simulink model "StratifiedHotWaterStorageTank"  (R2025a)
settings: Solver=VariableStepAuto  StartTime=0.0  StopTime=3600  RelTol=1e-3  AbsTol=1e-3
PreLoadFcn:
  | tankHeight = 1.6;
  | tankVolume = 0.2;
  | numberLayers = 8;
  | upwardConvectionCoeff = 50000;
  | downwardConvectionCoeff = 5;
libraries: fl_lib x30, nesl_utility x5, SimscapeFluids_lib x1
CloseFcn:
  | try, close(h1_StratifiedHotWaterStorageTank), end
  | clear h1_StratifiedHotWaterStorageTank
  | try, close(h2_StratifiedHotWaterStorageTank), end
  | clear h2_StratifiedHotWaterStorageTank
  | 
  | clear simlog_StratifiedHotWaterStorageTank
  | clear tankVolume tankHeight numberLayers upwardConvectionCoeff downwardConvectionCoeff
Description:
  | Stratified Hot Water Storage Tank
settings Model: Creator=The MathWorks, Inc.  LastModifiedBy=The MathWorks, Inc.
settings SolverCC: AutoScaleAbsTol=off  MaxConsecutiveMinStep=3  AlgebraicLoopSolver=TrustRegion  MaxZcPerStep=1.0
settings DataIOCC: SaveOutput=off  SignalLogging=off  DSMLogging=off  SaveTime=off  ReturnWorkspaceOutputs=off
settings DebuggingCC: UnconnectedInputMsg=warning  UnconnectedOutputMsg=warning  UnconnectedLineMsg=warning  SymbolicDimsDataTypeCodeGenerationDiagnostic=none
settings ModelReferenceCC: EnableRefExpFcnMdlSchedulingChecks=on
settings SFSimCC: CustomCodeUndefinedFunction=UseInterfaceOnly
settings RTWCC: GPUComputeCapability=3.5  DLArmComputeVersion=19.05
settings SimscapeCC: SimscapeLogType=all  SimscapeLogSimulationStatistics=on  SimscapeLogName=simlog_StratifiedHotWaterStorageTank  SimscapeLogLimitData=off  SimscapeLogDataHistory=10000.0

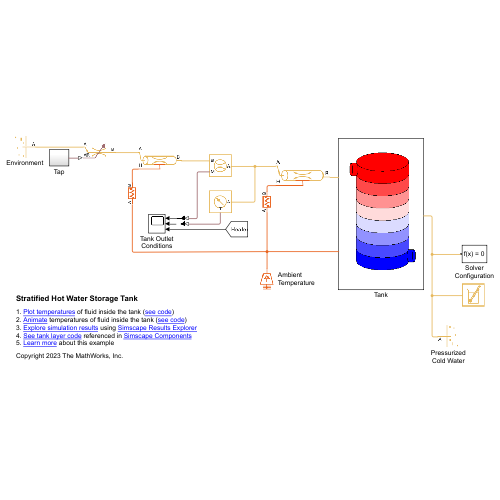
[thumbnail: Simulink's stored preview of the top-level diagram]
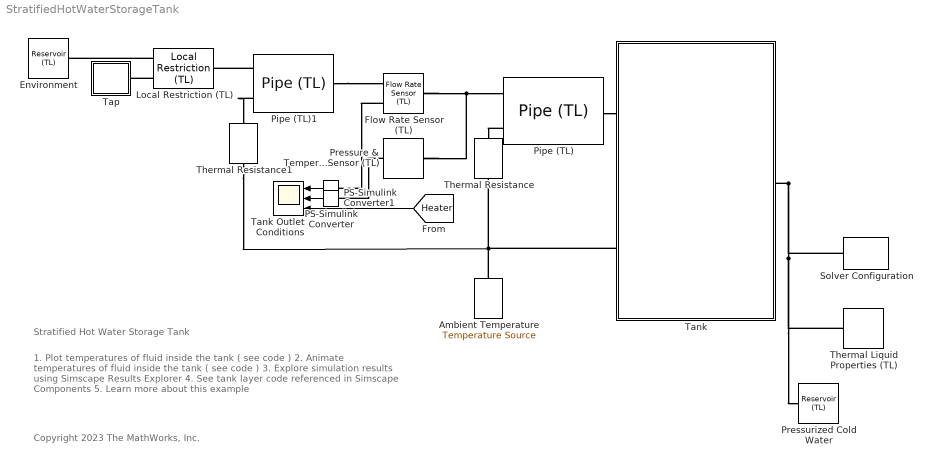
== system StratifiedHotWaterStorageTank ==
  note: 1. Plot temperatures of fluid inside the tank ( see code )
      | 2. Animate temperatures of fluid inside the tank ( see code )
      | 3. Explore simulation results using Simscape Results Explorer
      | 4. See tank layer code referenced in Simscape Components
      | 5. Learn more about this example
  note: Stratified Hot Water Storage Tank
  note: Copyright 2023 The MathWorks, Inc.
  Ambient Temperature : fl_lib/Thermal/Thermal Sources/Temperature Source  temperature=20 degC
  Environment : fl_lib/Thermal Liquid/Elements/Reservoir (TL)  pressure_spec=foundation.enum.pressure_spec.atmospheric  reservoir_pressure=0.101325 MPa  reservoir_temperature=20 degC  area=pi*0.02^2/4 m^2
  Flow Rate Sensor (TL) : fl_lib/Thermal Liquid/Sensors/Flow Rate Sensor (TL)  mass_flow_measure=true  volumetric_flow_measure=false  energy_flow_measure=false
      settings: InternalSimscapePortConfiguration="{\"Bottom\":[],\"Left\":[{\"id\":\"A\",\"label\":\"A\",\"type\":\"foundation.thermal_liquid.thermal_liquid\"}],\"Right\":[{\"id\":\"B\",\"label\":\"B\",\"type\":\"foundation.thermal_liquid.thermal_liquid\"},{\"id\":\"M\",\"label\":\"M\",\"type\":\"output\"}],\"Top\":[]}"
  Local Restriction (TL) : fl_lib/Thermal Liquid/Elements/Local Restriction (TL)  restriction_type=foundation.enum.restriction_type.variable  restriction_area=0.001 m^2  min_area=1e-10 m^2  max_area=7e-6 m^2  area=pi*0.02^2/4 m^2  Cd=0.64  Re_c=150  pressure_recovery=true
      settings: InternalSimscapePortConfiguration="{\"Bottom\":[],\"Left\":[{\"id\":\"A\",\"label\":\"A\",\"type\":\"foundation.thermal_liquid.thermal_liquid\"},{\"id\":\"area_in\",\"label\":\"AR\",\"type\":\"input\"}],\"Right\":[{\"id\":\"B\",\"label\":\"B\",\"type\":\"foundation.thermal_liquid.thermal_liquid\"}],\"Top\":[]}"
  PS-Simulink Converter : nesl_utility/PS-Simulink Converter  PhysicalDomain=network_engine_domain  SubClassName=ps_output  LeftPortType=input  RightPortType=output  PseudoPeriodic=off  Frequencies=[]  VectorFormat=inherit  Unit=inherit  AffineConversion=off
  PS-Simulink Converter1 : nesl_utility/PS-Simulink Converter  PhysicalDomain=network_engine_domain  SubClassName=ps_output  LeftPortType=input  RightPortType=output  PseudoPeriodic=off  Frequencies=[]  VectorFormat=inherit  Unit=degC  AffineConversion=on
  Pipe (TL) : fl_lib/Thermal Liquid/Elements/Pipe (TL)  length=10 m  area=pi*0.02^2/4 m^2  Dh=0.02 m  length_add=1 m  roughness=15e-6 m  Re_lam=2000  Re_tur=3000  shape_factor=64  Nu_lam=3.66  dynamic_compressibility=true  inertia=false  p0=0.101325 MPa  T0=20 degC  mdot0=0 kg/s  p_nominal=0.101325 MPa  T_nominal=293.15 K
  Pipe (TL)1 : fl_lib/Thermal Liquid/Elements/Pipe (TL)  length=0.1 m  area=pi*0.02^2/4 m^2  Dh=0.02 m  length_add=1 m  roughness=15e-6 m  Re_lam=2000  Re_tur=3000  shape_factor=64  Nu_lam=3.66  dynamic_compressibility=true  inertia=false  p0=0.101325 MPa  T0=20 degC  mdot0=0 kg/s  p_nominal=0.101325 MPa  T_nominal=293.15 K
  Pressure & Temperature Sensor (TL) : fl_lib/Thermal Liquid/Sensors/Pressure & Temperature Sensor (TL)  reference=foundation.enum.MeasurementReference.absolute  pressure=false  pressure_spec=foundation.enum.PressureMeasementSpec.Absolute  temperature=true
      settings: InternalSimscapePortConfiguration="{\"Bottom\":[{\"id\":\"T\",\"label\":\"T\",\"type\":\"output\"}],\"Left\":[{\"id\":\"A\",\"label\":\"A\",\"type\":\"foundation.thermal_liquid.thermal_liquid\"}],\"Right\":[],\"Top\":[]}"
  Pressurized Cold Water : fl_lib/Thermal Liquid/Elements/Reservoir (TL)  pressure_spec=foundation.enum.pressure_spec.specified  reservoir_pressure=0.3 MPa  reservoir_temperature=10 degC  area=pi*0.02^2/4 m^2
  Solver Configuration : nesl_utility/Solver Configuration  PhysicalDomain=network_engine_domain  SubClassName=solver  LeftPortType=input  RightPortType=generic  Tones=[]  Harmonics=[]  SimulateNoise=off  Profile=off  UseLocalSampling=off  EnableSwitchedLinearOptims=on  FrequencyDomain=off  UseCCode=off  RelTol=0.001  AbsTol=1e-06  MinStep=1e-09  ToWorkspace=off  RevertToSquareIcSolve=off  NumHomotopyIterations=100  PhasorMode=off  PhasorModeNumHarmonics=1  ConsistencySolver=NEWTON_XTOL_AFTER_FTOL  IndexReductionMethod=DerivativeReplacement  DoDC=off  ResidualTolerance=1e-09  ConsistencyTolSource=GLOBAL  ConsistencyAbsTol=0.001  ConsistencyRelTol=0.001  ConsistencyTolFactor=0.001  UseLocalSolver=off  LocalSolverChoice=NE_BACKWARD_EULER_ADVANCER  ResolveIndetEquations=on  FunctionEvalNumThread=1  LocalSolverSampleTime=0.001  DoFixedCost=off  MaxNonlinIter=3  MaxModeIter=2  ComputeImpulses=off  ImpulseIterations=2  LinearAlgebra=auto  LinearAlgebraNumThread=0  EquationFormulation=NE_TIME_EF  DelaysMemoryBudget=1024  AutomaticFiltering=on  FilteringTimeConstant=0.001  PartitionStorageMethod=AS_NEEDED  PartitionMemoryBudget=1024  PartitionMethod=ROBUST  MultibodyUseLocalSolver=off  MultibodyLocalSolverChoice=ODE1  MultibodyLocalSolverSampleTime=0.001
  Tank : Subsystem
      mask Display: image('StratifiedHotWaterStorageTank.png'); % Use "Edit Image" on toolstrip to change.
  Tank Outlet Conditions : Scope  NumInputPorts=3
      settings: Title=Mass Flow Rate (kg/s)  ActiveDisplayYMinimum=-0.01084  ActiveDisplayYMaximum=0.09753
  Tap : Subsystem
  Thermal Liquid Properties (TL) : SimscapeFluids_lib/Thermal Liquid/Utilities/Thermal Liquid Properties (TL)  fluid_list=fluids.thermal_liquid.utilities.enum.thermal_liquid_fluid_list.water  concentration_param_EG=fluids.thermal_liquid.utilities.enum.thermal_liquid_concentration.volume_fraction  concentration_param_PG=fluids.thermal_liquid.utilities.enum.thermal_liquid_concentration.volume_fraction  c_mass_SW=3.5e-3  c_mass_EG=0.1  c_mass_PG=0.1  c_mass_GL=0.1  c_vol_EG=0.1  c_vol_PG=0.1  beta_const_EG=2.1791 GPa  beta_const_PG=2.1791 GPa  beta_const_GL=2.1791 GPa  p_min_EG=0.01 MPa  p_min_PG=0.01 MPa  p_min_GL=0.01 MPa  p_max_EG=50 MPa  p_max_PG=50 MPa  p_max_GL=50 MPa  p_atm=0.101325 MPa  properties_range_check=simscape.enum.assert.action.error
  Thermal Resistance : fl_lib/Thermal/Thermal Elements/Thermal Resistance  resistance=3.125 K/W  T_specify=off  T_priority=None  T=0 K  T_nominal_specify=off  T_nominal_value=1  T_nominal_unit=K  Q_specify=off  Q_priority=None  Q=0 W  Q_nominal_specify=off  Q_nominal_value=1  Q_nominal_unit=W
  Thermal Resistance1 : fl_lib/Thermal/Thermal Elements/Thermal Resistance  resistance=3.125 K/W  T_specify=off  T_priority=None  T=0 K  T_nominal_specify=off  T_nominal_value=1  T_nominal_unit=K  Q_specify=off  Q_priority=None  Q=0 W  Q_nominal_specify=off  Q_nominal_value=1  Q_nominal_unit=W
  wires:
  PS-Simulink Converter/1 -> Tank Outlet Conditions/1
  PS-Simulink Converter1/1 -> Tank Outlet Conditions/2
  [Heater] -> Tank Outlet Conditions/3
  connections:
  Tank/RConn1 -- Pressurized Cold Water/LConn1 -- Thermal Liquid Properties (TL)/RConn1 -- Solver Configuration/RConn1
  Pipe (TL)/LConn2 -- Thermal Resistance/RConn1
  Ambient Temperature/LConn1 -- Tank/LConn2 -- Thermal Resistance/LConn1 -- Thermal Resistance1/LConn1
  Local Restriction (TL)/LConn2 -- Tap/RConn1
  Local Restriction (TL)/LConn1 -- Environment/LConn1
  Pipe (TL)/RConn1 -- Tank/LConn1
  Pressure & Temperature Sensor (TL)/RConn1 -- PS-Simulink Converter1/LConn1
  Flow Rate Sensor (TL)/RConn2 -- PS-Simulink Converter/LConn1
  Flow Rate Sensor (TL)/LConn1 -- Pressure & Temperature Sensor (TL)/LConn1 -- Pipe (TL)/LConn1
  Pipe (TL)1/RConn1 -- Flow Rate Sensor (TL)/RConn1
  Pipe (TL)1/LConn1 -- Local Restriction (TL)/RConn1
  Pipe (TL)1/LConn2 -- Thermal Resistance1/RConn1

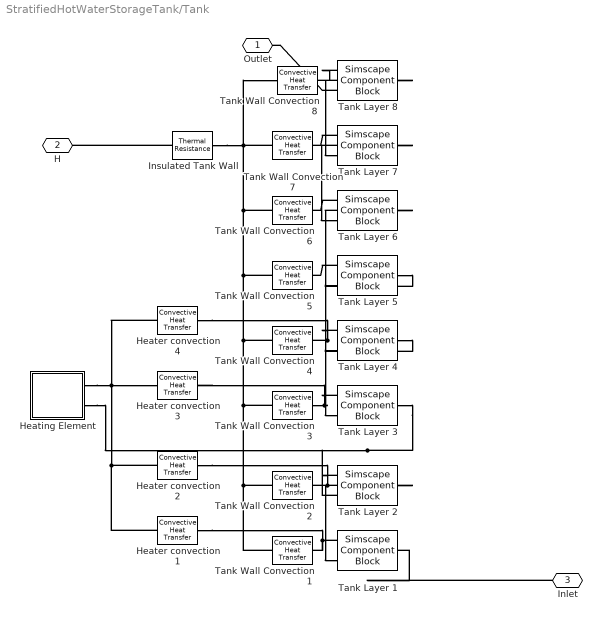
== system StratifiedHotWaterStorageTank/Tank ==
  Heater convection {1..4} (4 alike) : fl_lib/Thermal/Thermal Elements/Convective Heat Transfer  thermal_type=foundation.enum.constant_variable.constant  area=0.01 m^2  heat_tr_coeff=0.1 W/(K*m^2)  min_heat_tr_coeff=1e-3 W/(K*m^2)  T_specify=off  T_priority=None  T=0 K  T_nominal_specify=off  T_nominal_value=1  T_nominal_unit=K  Q_specify=off  Q_priority=None  Q=0 W  Q_nominal_specify=off  Q_nominal_value=1  Q_nominal_unit=W
  Heating Element : Subsystem
  Insulated Tank Wall : fl_lib/Thermal/Thermal Elements/Thermal Resistance  resistance=3.125 K/W  T_specify=off  T_priority=None  T=0 K  T_nominal_specify=off  T_nominal_value=1  T_nominal_unit=K  Q_specify=off  Q_priority=None  Q=0 W  Q_nominal_specify=off  Q_nominal_value=1  Q_nominal_unit=W
  Tank Layer 1 : SimscapeComponentBlock  SourceFile=StratifiedHotWaterStorageTankConstantVolume  ComponentPath=StratifiedHotWaterStorageTankConstantVolume  ComponentVariants="[\"StratifiedHotWaterStorageTankConstantVolume\"]"  ComponentVariantNames="[\"StratifiedHotWaterStorageTankConstantVolume\"]"  ClassName=StratifiedHotWaterStorageTankConstantVolume  SchemaVersion=1  volume=tankVolume/numberLayers m^3  elevation=tankHeight/numberLayers m  g=9.81 m/s^2  heat_tr_coeff_up=upwardConvectionCoeff W/(K*m^2)  heat_tr_coeff_down=downwardConvectionCoeff W/(K*m^2)  area_A=pi*0.02^2/4 m^2  area_B=tankVolume/tankHeight m^2  T_tol=1e-6 K  p_I_specify=on  p_I_priority=None  p_I=0.101325 MPa  p_I_nominal_specify=off  p_I_nominal_value=1  p_I_nominal_unit=MPa  T_I_specify=on  T_I_priority=High  T_I=40 degC  T_I_nominal_specify=off  T_I_nominal_value=1  T_I_nominal_unit=K  u_I_specify=off  u_I_priority=None  u_I=83.906 kJ/kg  u_I_nominal_specify=off  u_I_nominal_value=1  u_I_nominal_unit=kJ/kg  rho_I_specify=off  rho_I_priority=None  rho_I=998.21 kg/m^3  rho_I_nominal_specify=off  rho_I_nominal_value=1  rho_I_nominal_unit=kg/m^3
      settings: CopyFcn=simscape.sscblock.internal.componentBlockCallback(gcbh,'COPY')  PreCopyFcn=simscape.sscblock.internal.componentBlockCallback(gcbh,'PRECOPY')  PreDeleteFcn=simscape.sscblock.internal.componentBlockCallback(gcbh,'PREDELETE')  InternalSimscapePortConfiguration="{\"Bottom\":[{\"id\":\"A\",\"label\":\"A\",\"type\":\"foundation.thermal_liquid.thermal_liquid\"}],\"Left\":[{\"id\":\"H\",\"label\":\"H\",\"type\":\"foundation.thermal.thermal\"}],\"Right\":[],\"Top\":[{\"id\":\"B\",\"label\":\"B\",\"type\":\"foundation.thermal_liquid.thermal_liquid\"}]}"
      mask Type: Vertical Constant Volume (TL)
  Tank Layer {2..7} (6 alike) : SimscapeComponentBlock  SourceFile=StratifiedHotWaterStorageTankConstantVolume  ComponentPath=StratifiedHotWaterStorageTankConstantVolume  ComponentVariants="[\"StratifiedHotWaterStorageTankConstantVolume\"]"  ComponentVariantNames="[\"StratifiedHotWaterStorageTankConstantVolume\"]"  ClassName=StratifiedHotWaterStorageTankConstantVolume  SchemaVersion=1  volume=tankVolume/numberLayers m^3  elevation=tankHeight/numberLayers m  g=9.81 m/s^2  heat_tr_coeff_up=upwardConvectionCoeff W/(K*m^2)  heat_tr_coeff_down=downwardConvectionCoeff W/(K*m^2)  area_A=tankVolume/tankHeight m^2  area_B=tankVolume/tankHeight m^2  T_tol=1e-6 K  p_I_specify=on  p_I_priority=None  p_I=0.101325 MPa  p_I_nominal_specify=off  p_I_nominal_value=1  p_I_nominal_unit=MPa  T_I_specify=on  T_I_priority=High  T_I=40 degC  T_I_nominal_specify=off  T_I_nominal_value=1  T_I_nominal_unit=K  u_I_specify=off  u_I_priority=None  u_I=83.906 kJ/kg  u_I_nominal_specify=off  u_I_nominal_value=1  u_I_nominal_unit=kJ/kg  rho_I_specify=off  rho_I_priority=None  rho_I=998.21 kg/m^3  rho_I_nominal_specify=off  rho_I_nominal_value=1  rho_I_nominal_unit=kg/m^3
      settings: CopyFcn=simscape.sscblock.internal.componentBlockCallback(gcbh,'COPY')  PreCopyFcn=simscape.sscblock.internal.componentBlockCallback(gcbh,'PRECOPY')  PreDeleteFcn=simscape.sscblock.internal.componentBlockCallback(gcbh,'PREDELETE')  InternalSimscapePortConfiguration="{\"Bottom\":[{\"id\":\"A\",\"label\":\"A\",\"type\":\"foundation.thermal_liquid.thermal_liquid\"}],\"Left\":[{\"id\":\"H\",\"label\":\"H\",\"type\":\"foundation.thermal.thermal\"}],\"Right\":[],\"Top\":[{\"id\":\"B\",\"label\":\"B\",\"type\":\"foundation.thermal_liquid.thermal_liquid\"}]}"
      mask Type: Vertical Constant Volume (TL)
  Tank Layer 8 : SimscapeComponentBlock  SourceFile=StratifiedHotWaterStorageTankConstantVolume  ComponentPath=StratifiedHotWaterStorageTankConstantVolume  ComponentVariants="[\"StratifiedHotWaterStorageTankConstantVolume\"]"  ComponentVariantNames="[\"StratifiedHotWaterStorageTankConstantVolume\"]"  ClassName=StratifiedHotWaterStorageTankConstantVolume  SchemaVersion=1  volume=tankVolume/numberLayers m^3  elevation=tankHeight/numberLayers m  g=9.81 m/s^2  heat_tr_coeff_up=upwardConvectionCoeff W/(K*m^2)  heat_tr_coeff_down=downwardConvectionCoeff W/(K*m^2)  area_A=tankVolume/tankHeight m^2  area_B=pi*0.02^2/4 m^2  T_tol=1e-6 K  p_I_specify=on  p_I_priority=None  p_I=0.101325 MPa  p_I_nominal_specify=off  p_I_nominal_value=1  p_I_nominal_unit=MPa  T_I_specify=on  T_I_priority=High  T_I=40 degC  T_I_nominal_specify=off  T_I_nominal_value=1  T_I_nominal_unit=K  u_I_specify=off  u_I_priority=None  u_I=83.906 kJ/kg  u_I_nominal_specify=off  u_I_nominal_value=1  u_I_nominal_unit=kJ/kg  rho_I_specify=off  rho_I_priority=None  rho_I=998.21 kg/m^3  rho_I_nominal_specify=off  rho_I_nominal_value=1  rho_I_nominal_unit=kg/m^3
      settings: CopyFcn=simscape.sscblock.internal.componentBlockCallback(gcbh,'COPY')  PreCopyFcn=simscape.sscblock.internal.componentBlockCallback(gcbh,'PRECOPY')  PreDeleteFcn=simscape.sscblock.internal.componentBlockCallback(gcbh,'PREDELETE')  InternalSimscapePortConfiguration="{\"Bottom\":[{\"id\":\"A\",\"label\":\"A\",\"type\":\"foundation.thermal_liquid.thermal_liquid\"}],\"Left\":[{\"id\":\"H\",\"label\":\"H\",\"type\":\"foundation.thermal.thermal\"}],\"Right\":[],\"Top\":[{\"id\":\"B\",\"label\":\"B\",\"type\":\"foundation.thermal_liquid.thermal_liquid\"}]}"
      mask Type: Vertical Constant Volume (TL)
  Tank Wall Convection {1..8} (8 alike) : fl_lib/Thermal/Thermal Elements/Convective Heat Transfer  thermal_type=foundation.enum.constant_variable.constant  area=0.2*0.2*pi m^2  heat_tr_coeff=20 W/(K*m^2)  min_heat_tr_coeff=1e-3 W/(K*m^2)  T_specify=off  T_priority=None  T=0 K  T_nominal_specify=off  T_nominal_value=1  T_nominal_unit=K  Q_specify=off  Q_priority=None  Q=0 W  Q_nominal_specify=off  Q_nominal_value=1  Q_nominal_unit=W
  Outlet : PMIOPort  Side=Left
  H : PMIOPort  Port=2  Side=Left
  Inlet : PMIOPort  Port=3  Side=Right
  connections:
  Tank Layer 2/RConn1 -- Tank Layer 1/LConn2
  Tank Layer 4/RConn1 -- Tank Layer 3/LConn2
  Tank Layer 7/LConn1 -- Tank Wall Convection 7/RConn1
  Tank Layer 5/RConn1 -- Tank Layer 4/LConn2
  Tank Layer 8/RConn1 -- Tank Layer 7/LConn2
  Tank Layer 6/LConn1 -- Tank Wall Convection 6/RConn1
  Heater convection 2/RConn1 -- Tank Layer 2/LConn1 -- Tank Wall Convection 2/RConn1
  Tank Wall Convection 4/LConn1 -- Tank Wall Convection 5/LConn1 -- Tank Wall Convection 6/LConn1 -- Tank Wall Convection 7/LConn1 -- Insulated Tank Wall/RConn1 -- Tank Wall Convection 8/LConn1 -- Tank Wall Convection 1/LConn1 -- Tank Wall Convection 2/LConn1 -- Tank Wall Convection 3/LConn1
  Tank Layer 6/RConn1 -- Tank Layer 5/LConn2
  Heating Element/RConn2 -- Tank Layer 3/RConn1 -- Tank Layer 2/LConn2
  Tank Layer 8/LConn1 -- Tank Wall Convection 8/RConn1
  Tank Layer 1/LConn1 -- Tank Wall Convection 1/RConn1 -- Heater convection 1/RConn1
  Inlet/RConn1 -- Tank Layer 1/RConn1
  Tank Layer 5/LConn1 -- Tank Wall Convection 5/RConn1
  Insulated Tank Wall/LConn1 -- H/RConn1
  Tank Layer 7/RConn1 -- Tank Layer 6/LConn2
  Heater convection 4/RConn1 -- Tank Layer 4/LConn1 -- Tank Wall Convection 4/RConn1
  Tank Layer 8/LConn2 -- Outlet/RConn1
  Tank Wall Convection 3/RConn1 -- Tank Layer 3/LConn1 -- Heater convection 3/RConn1
  Heating Element/RConn1 -- Heater convection 1/LConn1 -- Heater convection 2/LConn1 -- Heater convection 4/LConn1 -- Heater convection 3/LConn1

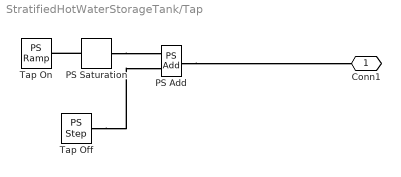
== system StratifiedHotWaterStorageTank/Tap ==
  PS Add : fl_lib/Physical Signals/Functions/PS Add
  PS Saturation : fl_lib/Physical Signals/Nonlinear Operators/PS Saturation  upper_limit=1  lower_limit=0  ZeroCross=true
  Tap Off : fl_lib/Physical Signals/Sources/PS Step  step_time=1560 s  initial_value=0  final_value=-1
  Tap On : fl_lib/Physical Signals/Sources/PS Ramp  slope=1 1/s  start_time=60 s  initial_output=0  ZeroCross=true
  Conn1 : PMIOPort  Side=Right
  connections:
  Tap Off/RConn1 -- PS Add/LConn2
  PS Saturation/LConn1 -- Tap On/RConn1
  PS Saturation/RConn1 -- PS Add/LConn1
  PS Add/RConn1 -- Conn1/RConn1

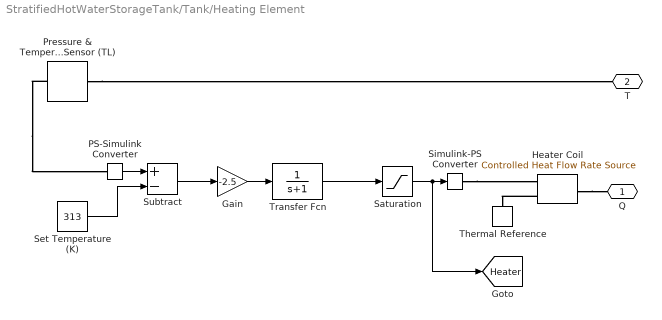
== system StratifiedHotWaterStorageTank/Tank/Heating Element ==
  Gain : Gain  Gain=-2.5
  Heater Coil : fl_lib/Thermal/Thermal Sources/Controlled Heat Flow Rate Source
  PS-Simulink Converter : nesl_utility/PS-Simulink Converter  PhysicalDomain=network_engine_domain  SubClassName=ps_output  LeftPortType=input  RightPortType=output  PseudoPeriodic=off  Frequencies=[]  VectorFormat=inherit  Unit=K  AffineConversion=off
  Pressure & Temperature Sensor (TL) : fl_lib/Thermal Liquid/Sensors/Pressure & Temperature Sensor (TL)  reference=foundation.enum.MeasurementReference.absolute  pressure=false  pressure_spec=foundation.enum.PressureMeasementSpec.Absolute  temperature=true
      settings: InternalSimscapePortConfiguration="{\"Bottom\":[{\"id\":\"T\",\"label\":\"T\",\"type\":\"output\"}],\"Left\":[{\"id\":\"A\",\"label\":\"A\",\"type\":\"foundation.thermal_liquid.thermal_liquid\"}],\"Right\":[],\"Top\":[]}"
  Saturation : Saturate  UpperLimit=2.5  LowerLimit=0
  Set Temperature (K) : Constant  Value=313
  Simulink-PS Converter : nesl_utility/Simulink-PS Converter  PhysicalDomain=network_engine_domain  SubClassName=ps_input  LeftPortType=input  RightPortType=output  PseudoPeriodic=off  Frequencies=[]  NoiseDistribution=none  NoiseParameters=[]  Unit=kW  AffineConversion=off  FilteringAndDerivatives=provide  SimscapeFilterOrder=1  InputFilterTimeConstant=0.001  UdotUserProvided=0
  Subtract : Sum  Inputs=+-
  Thermal Reference : fl_lib/Thermal/Thermal Elements/Thermal Reference
  Transfer Fcn : TransferFcn  Denominator=[1 1]
  Q : PMIOPort  Side=Right
  T : PMIOPort  Port=2  Side=Right
  tag scope: Heater=global
  wires:
  PS-Simulink Converter/1 -> Subtract/1
  Set Temperature (K)/1 -> Subtract/2
  Saturation/1 -> [Heater], Simulink-PS Converter/1
  Gain/1 -> Transfer Fcn/1
  Subtract/1 -> Gain/1
  Transfer Fcn/1 -> Saturation/1
  connections:
  Pressure & Temperature Sensor (TL)/LConn1 -- T/RConn1
  Heater Coil/LConn1 -- Q/RConn1
  Heater Coil/RConn2 -- Thermal Reference/LConn1
  Pressure & Temperature Sensor (TL)/RConn1 -- PS-Simulink Converter/LConn1
  Simulink-PS Converter/RConn1 -- Heater Coil/RConn1
